simulink model "fft_biplex_real_4x_dsp48_opt_test"  (Simulink 7.4)
settings: Solver=VariableStepDiscrete  StartTime=0.0  StopTime=128  RelTol=1e-3
libraries: xbsIndex_r4 x620, casper_library_misc x24, casper_library_delays x6, casper_library_ffts_twiddle x1, simulink x1
(part 1 of 7)
settings Model: Creator=User  LastModifiedBy=wjm
settings OptimizationCC: InitFltsAndDblsToZero=on
settings DebuggingCC: SaveWithDisabledLinksMsg=none  SaveWithParameterizedLinksMsg=none

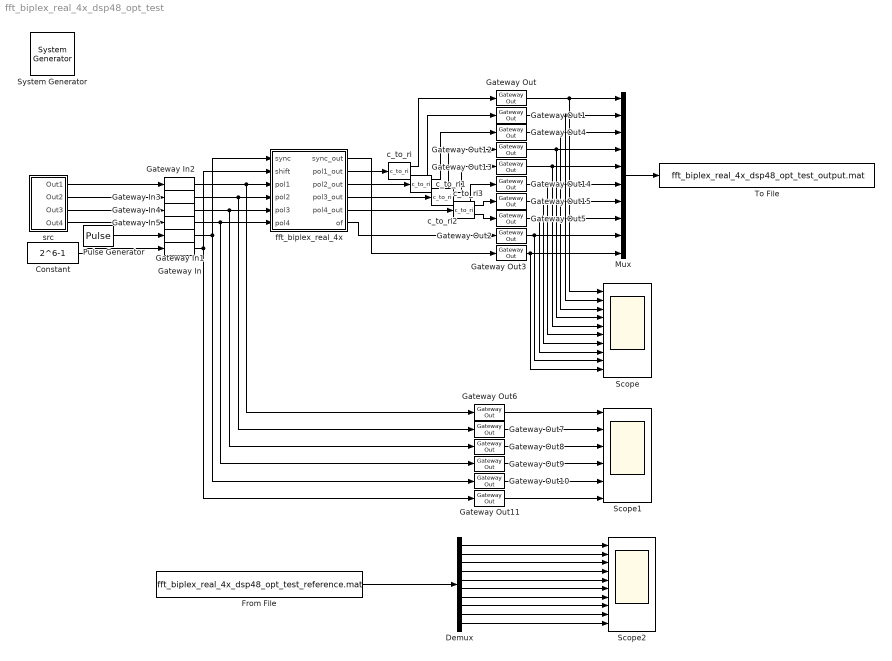
== system fft_biplex_real_4x_dsp48_opt_test ==
  " System Generator" : xbsIndex_r4/ System Generator  Tag=genX  SystemSampleTime=-1  xilinxfamily=virtex5  part=xc5vsx95t  speed=-1  package=ff1136  synthesis_tool=XST  clock_wrapper=Clock Enables  directory=./netlist  testbench=off  simulink_period=1  sysclk_period=100  dcm_input_clock_period=100  incr_netlist=off  trim_vbits=Everywhere in SubSystem  dbl_ovrd=According to Block Masks  core_generation=According to Block Masks  run_coregen=off  deprecated_control=off  eval_field=0  block_type=sysgen
      settings: block_version=10.1.1
  Constant : Constant  Value=2^6-1  OutDataType=sfix(16)  OutScaling=2^0
  Demux : Demux  Outputs=10
  From File : FromFile  FileName=fft_biplex_real_4x_dsp48_opt_test_reference.mat  SampleTime=1
  Gateway In : xbsIndex_r4/Gateway In  arith_type=Unsigned  n_bits=6  bin_pt=0  quantization=Truncate  overflow=Wrap  period=1  dbl_ovrd=off  timing_constraint=None  locs_specified=off  LOCs={}  hdl_port=on  block_type=gatewayin
      settings: infoedit="Gateway in block.  Converts inputs of type Simulink integer, double and fixed point to  Xilinx fixed point type.<P><P>Hardware notes:  In hardware these blocks become top level input ports."  block_version=10.1.1
  Gateway In1 : xbsIndex_r4/Gateway In  arith_type=Boolean  n_bits=16  bin_pt=14  quantization="Round  (unbiased: +/- Inf)"  overflow=Saturate  period=1  dbl_ovrd=off  timing_constraint=None  locs_specified=off  LOCs={}  hdl_port=on  block_type=gatewayin
      settings: infoedit="Gateway in block.  Converts inputs of type Simulink integer, double and fixed point to  Xilinx fixed point type.<P><P>Hardware notes:  In hardware these blocks become top level input ports."  block_version=10.1.1
  Gateway In{2..5} (4 alike) : xbsIndex_r4/Gateway In  arith_type="Signed  (2's comp)"  n_bits=8  bin_pt=7  quantization=Truncate  overflow=Wrap  period=1  dbl_ovrd=off  timing_constraint=None  locs_specified=off  LOCs={}  hdl_port=on  block_type=gatewayin
      settings: infoedit="Gateway in block.  Converts inputs of type Simulink integer, double and fixed point to  Xilinx fixed point type.<P><P>Hardware notes:  In hardware these blocks become top level input ports."  block_version=10.1.1
  Gateway Out{,1..15} (16 alike) : xbsIndex_r4/Gateway Out  hdl_port=on  timing_constraint=None  locs_specified=off  LOCs={}  block_type=gatewayout
      settings: infoedit="Gateway out block.  Converts Xilinx fixed point inputs into ouputs of type Simulink integer, double, or fixed point.<P><P>Hardware notes:  In hardware these blocks become top level output ports or are discarded, depending on how they are configured."  block_version=10.1.1
  Mux : Mux  Inputs=10
  Pulse Generator : DiscretePulseGenerator  Amplitude=1  Period=2^5  PulseWidth=1  PhaseDelay=13  SampleTime=1
  Scope : Scope  NumInputPorts=10
      settings: TimeRange=256  YMin=-5~-5~-5~-5~-1~-5~-5~-5~-5~-5  YMax=5~5~5~5~2~5~5~5~5~5
  Scope1 : Scope  NumInputPorts=6
      settings: YMin=-5~-5~-5~-5~-5~-5  YMax=5~5~5~5~5~5
  Scope2 : Scope  NumInputPorts=10
      settings: TimeRange=256  YMin=-5~-5~-5~-5~-1~-5~-5~-5~-5~-5  YMax=5~5~5~5~2~5~5~5~5~5  SaveName=ScopeData2
  To File : ToFile  Filename=fft_biplex_real_4x_dsp48_opt_test_output.mat  MatrixName=output
  c_to_ri{,1..3} (4 alike) : casper_library_misc/c_to_ri  SystemSampleTime=-1  n_bits=8  bin_pt=7
      settings: AttributesFormatString=8_7 r/i
  fft_biplex_real_4x : Subsystem  AncestorBlock=casper_library_ffts/fft_biplex_real_4x  mask(fft_biplex_real_4x){FFTSize=3, input_bit_width=8, coeff_bit_width=8, add_latency=2, mult_latency=3, bram_latency=1, conv_latency=1, quantization=Truncate, overflow=Wrap, arch=Virtex5, opt_target=logic, coeffs_bit_limit=8, delays_bit_limit=8, specify_mult=on, mult_spec=[0                                      1                                      2], hardcode_shifts=off, shift_schedule=getfield( getfield( get_param( gcb,'UserData' ), 'parameters'),'shift_schedule'), dsp48_adders=on}
      mask prompts: FFTSize "Size of FFT: (2^? pts)"; input_bit_width "Input/Output Bit Width"; coeff_bit_width "Coefficient Bit Width"; add_latency "Add Latency"; mult_latency "Mult Latency"; bram_latency "BRAM Latency"; conv_latency "Convert latency"; quantization "Quantization Behavior"; overflow "Overflow Behavior"; arch "Architecture"; opt_target "Use less"; coeffs_bit_limit "Number bits above which to store stage's coefficients in BRAM (2^? bits)"; delays_bit_limit "Number bits above which to implement stage's delays in BRAM (2^? bits)"; specify_mult "Specify multiplier use (behavioral HDL if not specified)"; mult_spec "Multiplier specification (0=core, 1=embedded, 2=behavioural) (left=1st stage)"; hardcode_shifts "Hardcode shift schedule"; shift_schedule "Shift schedule"; dsp48_adders "DSP48 adders in butterfly"
      mask help: A real-sampled biplex FFT, with output demuxed by 4.
      mask init:
      | fft_biplex_real_4x_init(gcb, ...
      |     'FFTSize', FFTSize, ...
      |     'input_bit_width', input_bit_width, ...
      |     'coeff_bit_width', coeff_bit_width, ...
      |     'add_latency', add_latency, ...
      |     'mult_latency', mult_latency, ...
      |     'bram_latency', bram_latency, ...
      |     'conv_latency', conv_latency, ...
      |     'quantization', quantization, ...
      |     'overflow', overflow, ...
      |     'arch', arch, ...
      |     'opt_target', opt_target, ...
      |     'coeffs_bit_limit', coeffs_bit_limit, ...
      |     'delays_bit_limit', delays_bit_limit, ...    
      |     'specify_mult', specify_mult, ...
      |     'mult_spec', mult_spec, ...
      |     'hardcode_shifts', hardcode_shifts, ...
      |     'shift_schedule', shift_schedule, ...
      |     'dsp48_adders', dsp48_adders);
      settings: AttributesFormatString=|
      | Virtex5
      | 3 stages
      | [8,8]
      | Truncate
      | Wrap
      mask Help: eval('xlWeb(''http://casper.berkeley.edu/wiki/Fft_biplex_real_4x'')')
      mask StyleString: edit,edit,edit,edit,edit,edit,edit,popup(Truncate|Round  (unbiased: +/- Inf)|Round  (unbiased: Even Values)),popup(Wrap|Saturate|Error),popup(Virtex2Pro|Virtex5),popup(logic|multipliers),edit,edit,checkbox,edit,checkbox,edit,checkbox
      mask CallbackString:
      | |||||||||fft_callback_arch(gcb);||||specify_mult = get_param(gcb, 'specify_mult');
      | set_param_state(gcb, 'mult_spec', specify_mult);||hardcode_shifts = get_param(gcb, 'hardcode_shifts');
      | set_param_state(gcb, 'shift_schedule', hardcode_shifts);||fft_callback_dsp48_adders(gcb);
      mask TabNameString: Basic,Basic,Basic,Latency,Latency,Latency,Latency,Implementation,Implementation,Implementation,Implementation,Implementation,Implementation,Implementation,Implementation,Implementation,Implementation,Implementation
  src : Subsystem
  wires:
  Gateway In/1 -> Gateway Out11/1, fft_biplex_real_4x/2(shift)
  Pulse Generator/1 -> Gateway In1/1
  Gateway In1/1 -> Gateway Out10/1, fft_biplex_real_4x/1(sync)
  src/1(Out1) -> Gateway In2/1
  src/2(Out2) -> Gateway In3/1
  src/3(Out3) -> Gateway In4/1
  src/4(Out4) -> Gateway In5/1
  Gateway In2/1 -> Gateway Out6/1, fft_biplex_real_4x/3(pol1)
  Gateway In3/1 -> Gateway Out7/1, fft_biplex_real_4x/4(pol2)
  Gateway In4/1 -> Gateway Out8/1, fft_biplex_real_4x/5(pol3)
  Gateway In5/1 -> Gateway Out9/1, fft_biplex_real_4x/6(pol4)
  Gateway Out6/1 -> Scope1/1
  Gateway Out7/1 -> Scope1/2
  Gateway Out8/1 -> Scope1/3
  Gateway Out9/1 -> Scope1/4
  Gateway Out10/1 -> Scope1/5
  Gateway Out11/1 -> Scope1/6
  Constant/1 -> Gateway In/1
  Mux/1 -> To File/1
  c_to_ri/1 -> Gateway Out/1
  c_to_ri/2 -> Gateway Out1/1
  c_to_ri1/1 -> Gateway Out4/1
  c_to_ri1/2 -> Gateway Out12/1
  c_to_ri2/1 -> Gateway Out13/1
  c_to_ri2/2 -> Gateway Out14/1
  c_to_ri3/1 -> Gateway Out15/1
  c_to_ri3/2 -> Gateway Out5/1
  Gateway Out/1 -> Scope/1, Mux/1
  Gateway Out1/1 -> Scope/2, Mux/2
  Gateway Out4/1 -> Scope/3, Mux/3
  Gateway Out12/1 -> Scope/4, Mux/4
  Gateway Out13/1 -> Scope/5, Mux/5
  Gateway Out14/1 -> Scope/6, Mux/6
  Gateway Out15/1 -> Scope/7, Mux/7
  Gateway Out5/1 -> Scope/8, Mux/8
  Gateway Out2/1 -> Scope/9, Mux/9
  Gateway Out3/1 -> Scope/10, Mux/10
  Demux/1 -> Scope2/1
  Demux/2 -> Scope2/2
  Demux/3 -> Scope2/3
  Demux/4 -> Scope2/4
  Demux/5 -> Scope2/5
  Demux/6 -> Scope2/6
  Demux/7 -> Scope2/7
  Demux/8 -> Scope2/8
  Demux/9 -> Scope2/9
  Demux/10 -> Scope2/10
  From File/1 -> Demux/1
  fft_biplex_real_4x/2(pol1_out) -> c_to_ri/1
  fft_biplex_real_4x/3(pol2_out) -> c_to_ri1/1
  fft_biplex_real_4x/4(pol3_out) -> c_to_ri2/1
  fft_biplex_real_4x/5(pol4_out) -> c_to_ri3/1
  fft_biplex_real_4x/6(of) -> Gateway Out2/1
  fft_biplex_real_4x/1(sync_out) -> Gateway Out3/1

== system fft_biplex_real_4x_dsp48_opt_test/fft_biplex_real_4x ==
  sync : Inport  OutDataType=sfix(16)  OutScaling=2^0
  shift : Inport  Port=2  OutDataType=sfix(16)  OutScaling=2^0
  pol1 : Inport  Port=3  OutDataType=sfix(16)  OutScaling=2^0
  pol2 : Inport  Port=4  OutDataType=sfix(16)  OutScaling=2^0
  pol3 : Inport  Port=5  OutDataType=sfix(16)  OutScaling=2^0
  pol4 : Inport  Port=6  OutDataType=sfix(16)  OutScaling=2^0
  bi_real_unscr_4x : Subsystem  AncestorBlock=casper_library_ffts_internal/bi_real_unscr_4x  mask(bi_real_unscr_4x){FFTSize=3, n_bits=8, add_latency=2, conv_latency=1, bram_latency=1, bram_map=off, bram_delays=off, dsp48_adders=on}
      mask prompts: FFTSize "Size of FFT (2^?):"; n_bits "Sample Bit Width"; add_latency "Add Latency"; conv_latency "Convert Latency"; bram_latency "BRAM Latency"; bram_map "Use BlockRAM for Map"; bram_delays "Use BlockRAM for Delays"; dsp48_adders "Use DSP48s for adders"
      mask help: FFT internal block.
      mask init:
      | bi_real_unscr_4x_init(gcb, ...
      |     'FFTSize', FFTSize, ...
      |     'n_bits', n_bits, ...
      |     'add_latency', add_latency, ...
      |     'conv_latency', conv_latency, ...
      |     'bram_latency', bram_latency, ...
      |     'bram_map', bram_map, ...
      |     'bram_delays', bram_delays, ...
      |     'dsp48_adders', dsp48_adders);
      mask TabNameString: Basic,Basic,Latency,Latency,Latency,Implementation,Implementation,Implementation
  biplex_core : Subsystem  AncestorBlock=casper_library_ffts/biplex_core  mask(biplex_core){FFTSize=3, input_bit_width=8, coeff_bit_width=8, add_latency=2, mult_latency=3, bram_latency=1, conv_latency=1, quantization=Truncate, overflow=Wrap, arch=Virtex5, opt_target=logic, coeffs_bit_limit=8, delays_bit_limit=8, specify_mult=on, mult_spec=[0                                      1                                      2], hardcode_shifts=off, shift_schedule=getfield( getfield( get_param( gcb,'UserData' ), 'parameters'),'shift_schedule'), dsp48_adders=on}
      mask prompts: FFTSize "Size of FFT: (2^? pts)"; input_bit_width "Input/Output Bit Width"; coeff_bit_width "Coefficient Bit Width"; add_latency "Add Latency"; mult_latency "Mult Latency"; bram_latency "BRAM Latency"; conv_latency "Convert latency"; quantization "Quantization Behavior"; overflow "Overflow Behavior"; arch "Architecture"; opt_target "Use less"; coeffs_bit_limit "Number bits above which to store stage's coefficients in BRAM (2^? bits)"; delays_bit_limit "Number bits above which to implent stage's delays in BRAM (2^? bits)"; specify_mult "Specify multiplier use (behavioural HDL if not specified)"; mult_spec "Multiplier specification (0=core, 1=embedded, 2=behavioural) (left=1st stage)"; hardcode_shifts "Hardcode shift schedule"; shift_schedule "Shift schedule"; dsp48_adders "Use DSP48s for adders"
      mask help: FFT internal block.
      mask init:
      | biplex_core_init(gcb,...
      |     'FFTSize', FFTSize,...
      |     'input_bit_width', input_bit_width,...
      |     'coeff_bit_width', coeff_bit_width,...
      |     'add_latency', add_latency,...
      |     'mult_latency', mult_latency,...
      |     'bram_latency', bram_latency,...
      |     'conv_latency', conv_latency, ...
      |     'quantization', quantization,...
      |     'overflow', overflow,...
      |     'arch', arch, ...
      |     'opt_target', opt_target, ...
      |     'coeffs_bit_limit', coeffs_bit_limit, ...
      |     'delays_bit_limit', delays_bit_limit, ...
      |     'specify_mult', specify_mult, ...
      |     'mult_spec', mult_spec, ...
      |     'hardcode_shifts', hardcode_shifts, ...
      |     'shift_schedule', shift_schedule, ...
      |     'dsp48_adders', dsp48_adders );
      settings: AttributesFormatString=|
      | 3 stages
      | reduce logic
      | Virtex5
      mask StyleString: edit,edit,edit,edit,edit,edit,edit,popup(Truncate|Round  (unbiased: +/- Inf)|Round  (unbiased: Even Values)),popup(Wrap|Saturate|Error),popup(Virtex2Pro|Virtex5),popup(logic|multipliers),edit,edit,checkbox,edit,checkbox,edit,checkbox
      mask CallbackString:
      | |||||||||fft_callback_arch(gcb);||||specify_mult = get_param(gcb, 'specify_mult');
      | set_param_state(gcb, 'mult_spec', specify_mult);||hardcode_shifts = get_param(gcb, 'hardcode_shifts');
      | set_param_state(gcb, 'shift_schedule', hardcode_shifts);||fft_callback_dsp48_adders(gcb);
      mask TabNameString: Basic,Basic,Basic,Latency,Latency,Latency,Latency,Implementation,Implementation,Implementation,Implementation,Implementation,Implementation,Implementation,Implementation,Implementation,Implementation,Implementation
  ri_to_c0 : Subsystem  AncestorBlock=casper_library_misc/ri_to_c
      mask Type: ri_to_c
      mask Description:
      | Concatenates real and imaginary inputs into a complex output.
      | Useful for simplifying interconnects.
      | See also: Complex to Real-Imag (c_to_ri)
      mask Help: eval('xlWeb(''http://casper.berkeley.edu/wiki/Ri_to_c'')')
  ri_to_c1 : Subsystem  AncestorBlock=casper_library_misc/ri_to_c
      mask Type: ri_to_c
      mask Description:
      | Concatenates real and imaginary inputs into a complex output.
      | Useful for simplifying interconnects.
      | See also: Complex to Real-Imag (c_to_ri)
      mask Help: eval('xlWeb(''http://casper.berkeley.edu/wiki/Ri_to_c'')')
  sync_out : Outport  OutDataType=sfix(16)  OutScaling=2^0
  pol1_out : Outport  Port=2  OutDataType=sfix(16)  OutScaling=2^0
  pol2_out : Outport  Port=3  OutDataType=sfix(16)  OutScaling=2^0
  pol3_out : Outport  Port=4  OutDataType=sfix(16)  OutScaling=2^0
  pol4_out : Outport  Port=5  OutDataType=sfix(16)  OutScaling=2^0
  of : Outport  Port=6  OutDataType=sfix(16)  OutScaling=2^0
  wires:
  pol1/1 -> ri_to_c0/1(re)
  pol2/1 -> ri_to_c0/2(im)
  pol3/1 -> ri_to_c1/1(re)
  pol4/1 -> ri_to_c1/2(im)
  sync/1 -> biplex_core/1(sync)
  shift/1 -> biplex_core/2(shift)
  ri_to_c0/1(c) -> biplex_core/3(pol1)
  ri_to_c1/1(c) -> biplex_core/4(pol2)
  biplex_core/1(sync_out) -> bi_real_unscr_4x/1(sync)
  biplex_core/2(out1) -> bi_real_unscr_4x/2(even)
  biplex_core/3(out2) -> bi_real_unscr_4x/3(odd)
  biplex_core/4(of) -> of/1
  bi_real_unscr_4x/1(sync_out) -> sync_out/1
  bi_real_unscr_4x/2(pol1_out) -> pol1_out/1
  bi_real_unscr_4x/3(pol2_out) -> pol2_out/1
  bi_real_unscr_4x/4(pol3_out) -> pol3_out/1
  bi_real_unscr_4x/5(pol4_out) -> pol4_out/1

== system fft_biplex_real_4x_dsp48_opt_test/src ==
  Band-Limited White Noise : simulink/Sources/Band-Limited White Noise  SystemSampleTime=-1  Cov=[0.001]  Ts=1  seed=[23341]
  Constant : Constant  Value=0  OutDataType=sfix(16)  OutScaling=2^0
  Pulse Generator1 : DiscretePulseGenerator  Amplitude=0.75  Period=2^4  PulseWidth=1  PhaseDelay=15  SampleTime=1
  Pulse Generator2 : DiscretePulseGenerator  Amplitude=0.75  Period=2^3  PulseWidth=1  PhaseDelay=16  SampleTime=1
  Sine Wave : Sin  SineType=Sample based  Amplitude=0.1  Bias=0  Frequency=1  Phase=0  Samples=8  SampleTime=1  Offset=0
  Out1 : Outport
  Out2 : Outport  Port=2
  Out3 : Outport  Port=3
  Out4 : Outport  Port=4
  wires:
  Pulse Generator1/1 -> Out1/1
  Constant/1 -> Out3/1
  Sine Wave/1 -> Out2/1
  Band-Limited White Noise/1 -> Out4/1

== system fft_biplex_real_4x_dsp48_opt_test/fft_biplex_real_4x/bi_real_unscr_4x ==
  sync : Inport
  even : Inport  Port=2
  odd : Inport  Port=3
  Constant0 : xbsIndex_r4/Constant  arith_type=Unsigned  const=2^(FFTSize-1)  n_bits=FFTSize  bin_pt=0  explicit_period=on  period=1  equ=P=C  opselect=C  inp2=PCIN>>17  opr=+  inp1=P  carry=CIN  dbl_ovrd=off  block_type=constant
      settings: block_version=11.4
  Constant1 : xbsIndex_r4/Constant  arith_type=Unsigned  const=0  n_bits=FFTSize  bin_pt=0  explicit_period=on  period=1  equ=P=C  opselect=C  inp2=PCIN>>17  opr=+  inp1=P  carry=CIN  dbl_ovrd=off  block_type=constant
      settings: block_version=11.4
  Counter0 : xbsIndex_r4/Counter  cnt_type=Free Running  cnt_to=Inf  operation=Up  start_count=0  cnt_by_val=1  arith_type=Unsigned  n_bits=FFTSize  bin_pt=0  load_pin=off  rst=on  en=off  explicit_period=on  period=1  dbl_ovrd=off  use_behavioral_HDL=off  implementation=Fabric  block_type=counter
      settings: block_version=11.4
  Delay : xbsIndex_r4/Delay  en=off  latency=1  dbl_ovrd=off  reg_retiming=off  block_type=delay
      settings: block_version=11.4
  Mux{0..3} (4 alike) : xbsIndex_r4/Mux  inputs=2  en=off  latency=1  precision=Full  arith_type=Unsigned  n_bits=16  bin_pt=14  quantization=Truncate  overflow=Wrap  dbl_ovrd=off  block_type=mux
      settings: block_version=11.4
  Relational0 : xbsIndex_r4/Relational  mode=a=b  en=off  latency=0  dbl_ovrd=off  block_type=relational
  Relational1 : xbsIndex_r4/Relational  mode=a=b  en=off  latency=0  dbl_ovrd=off  block_type=relational
  delay_srl0 : Subsystem  AncestorBlock=casper_library_delays/delay_srl  mask(delay_srl){DelayLen=2^(FFTSize-1)}
      mask prompts: DelayLen "Delay by:"
      mask help:
      | A delay block that uses slices (SRL16s) for its storage.
      |
      | It explicitly converts the first delay into a flip flop,
      | and lets XSG break up the remaining delays into a series
      | of SRL16+FF instances.
      |
      | This is advantageous because the setup time of an SRL is
      | longer than that of a flip flop.
      mask init:
      | if (DelayLen > 0),
      |     ff_delay = 1;
      |     srl_delay = DelayLen - 1;
      | else
      |     ff_delay = 0;
      |     srl_delay = 0;
      | end
      mask Help: eval('xlWeb(''http://casper.berkeley.edu/wiki/Delay_srl'')')
  delay_srl1 : Subsystem  AncestorBlock=casper_library_delays/delay_srl  mask(delay_srl){DelayLen=2^(FFTSize-1)}
      mask prompts: DelayLen "Delay by:"
      mask help:
      | A delay block that uses slices (SRL16s) for its storage.
      |
      | It explicitly converts the first delay into a flip flop,
      | and lets XSG break up the remaining delays into a series
      | of SRL16+FF instances.
      |
      | This is advantageous because the setup time of an SRL is
      | longer than that of a flip flop.
      mask init:
      | if (DelayLen > 0),
      |     ff_delay = 1;
      |     srl_delay = DelayLen - 1;
      | else
      |     ff_delay = 0;
      |     srl_delay = 0;
      | end
      mask Help: eval('xlWeb(''http://casper.berkeley.edu/wiki/Delay_srl'')')
  en_even : xbsIndex_r4/Constant  arith_type=Boolean  const=1  n_bits=1  bin_pt=0  explicit_period=on  period=1  equ=P=C  opselect=C  inp2=PCIN>>17  opr=+  inp1=P  carry=CIN  dbl_ovrd=off  block_type=constant
      settings: block_version=11.4
  en_odd : xbsIndex_r4/Constant  arith_type=Boolean  const=1  n_bits=1  bin_pt=0  explicit_period=on  period=1  equ=P=C  opselect=C  inp2=PCIN>>17  opr=+  inp1=P  carry=CIN  dbl_ovrd=off  block_type=constant
      settings: block_version=11.4
  en_out : xbsIndex_r4/Constant  arith_type=Boolean  const=1  n_bits=1  bin_pt=0  explicit_period=on  period=1  equ=P=C  opselect=C  inp2=PCIN>>17  opr=+  inp1=P  carry=CIN  dbl_ovrd=off  block_type=constant
      settings: block_version=11.4
  hilbert_dsp48e0 : Subsystem  AncestorBlock=casper_library_ffts_internal/hilbert_dsp48e  mask(sincos_dsp48e){BitWidth=n_bits, conv_latency=conv_latency}
      mask prompts: BitWidth "Bit Wdith"; conv_latency "Convert Latency"
      mask help:
      | FFT internal block.
      |
      | Computes (a+b*)/2 and (a-b*)/2i.
  hilbert_dsp48e1 : Subsystem  AncestorBlock=casper_library_ffts_internal/hilbert_dsp48e  mask(sincos_dsp48e){BitWidth=n_bits, conv_latency=conv_latency}
      mask prompts: BitWidth "Bit Wdith"; conv_latency "Convert Latency"
      mask help:
      | FFT internal block.
      |
      | Computes (a+b*)/2 and (a-b*)/2i.
  mirror_spectrum : Subsystem  AncestorBlock=casper_library_ffts_internal/mirror_spectrum  mask(mirror_spectrum){FFTSize=3, input_bitwidth=8, bram_latency=1, negate_latency=1}
      mask prompts: FFTSize "Size of FFT (2^?)"; input_bitwidth "Input Bit Width"; bram_latency "BRAM Latency"; negate_latency "Negate Latency"
      mask help: FFT internal block.
      mask TabNameString: Basic,Basic,Latency,Latency
  reorder_even : Subsystem  AncestorBlock=casper_library_reorder/reorder  mask(reorder){map=[0 2 1 3], n_inputs=1, bram_latency=bram_latency, map_latency=0, double_buffer=0, bram_map=off}
      mask prompts: map "Output Order:"; n_inputs "Number of inputs"; bram_latency "BRAM Latency"; map_latency "Map Latency"; double_buffer "Double Buffer"; bram_map "Use BlockRAM for Map"
      mask init:
      | reorder_init(gcb, ...
      |     'map', map, ...
      |     'n_inputs', n_inputs, ...
      |     'bram_latency', bram_latency, ...
      |     'map_latency', map_latency, ...
      |     'double_buffer', double_buffer, ...
      |     'bram_map', bram_map);
      settings: AttributesFormatString=order=2
      mask Help: eval('xlWeb(''http://casper.berkeley.edu/wiki/Reorder'')')
  reorder_odd : Subsystem  AncestorBlock=casper_library_reorder/reorder  mask(reorder){map=[3 1 2 0], n_inputs=1, bram_latency=bram_latency, map_latency=0, double_buffer=0, bram_map=off}
      mask prompts: map "Output Order:"; n_inputs "Number of inputs"; bram_latency "BRAM Latency"; map_latency "Map Latency"; double_buffer "Double Buffer"; bram_map "Use BlockRAM for Map"
      mask init: same as fft_biplex_real_4x_dsp48_opt_test/fft_biplex_real_4x/bi_real_unscr_4x/reorder_even
      settings: AttributesFormatString=order=2
      mask Help: eval('xlWeb(''http://casper.berkeley.edu/wiki/Reorder'')')
  reorder_out : Subsystem  AncestorBlock=casper_library_reorder/reorder  mask(reorder){map=[3 2 1 0], n_inputs=4, bram_latency=bram_latency, map_latency=0, double_buffer=0, bram_map=off}
      mask prompts: map "Output Order:"; n_inputs "Number of inputs"; bram_latency "BRAM Latency"; map_latency "Map Latency"; double_buffer "Double Buffer"; bram_map "Use BlockRAM for Map"
      mask init: same as fft_biplex_real_4x_dsp48_opt_test/fft_biplex_real_4x/bi_real_unscr_4x/reorder_even
      settings: AttributesFormatString=order=2
      mask Help: eval('xlWeb(''http://casper.berkeley.edu/wiki/Reorder'')')
  sync_delay_srl : Subsystem  AncestorBlock=casper_library_delays/delay_srl  mask(delay_srl){DelayLen=2^(FFTSize-1) + add_latency + conv_latency + 1}
      mask prompts: DelayLen "Delay by:"
      mask help:
      | A delay block that uses slices (SRL16s) for its storage.
      |
      | It explicitly converts the first delay into a flip flop,
      | and lets XSG break up the remaining delays into a series
      | of SRL16+FF instances.
      |
      | This is advantageous because the setup time of an SRL is
      | longer than that of a flip flop.
      mask init:
      | if (DelayLen > 0),
      |     ff_delay = 1;
      |     srl_delay = DelayLen - 1;
      | else
      |     ff_delay = 0;
      |     srl_delay = 0;
      | end
      mask Help: eval('xlWeb(''http://casper.berkeley.edu/wiki/Delay_srl'')')
  sync_out : Outport
  pol1_out : Outport  Port=2
  pol2_out : Outport  Port=3
  pol3_out : Outport  Port=4
  pol4_out : Outport  Port=5
  wires:
  sync/1 -> reorder_even/1(sync), reorder_odd/1(sync)
  en_even/1 -> reorder_even/2(en)
  even/1 -> reorder_even/3(din0)
  en_odd/1 -> reorder_odd/2(en)
  odd/1 -> reorder_odd/3(din0)
  reorder_odd/3(dout0) -> Delay/1
  reorder_even/1(sync_out) -> Counter0/1, sync_delay_srl/1(in)
  Constant0/1 -> Relational0/1
  Counter0/1 -> Relational0/2, Relational1/1
  Constant1/1 -> Relational1/2
  Relational0/1 -> Mux0/1, Mux3/1
  Relational1/1 -> Mux1/1, Mux2/1
  reorder_even/3(dout0) -> Mux0/2, Mux1/3, Mux2/2, Mux3/3
  Delay/1 -> Mux0/3, Mux1/2, Mux2/3, Mux3/2
  Mux0/1 -> hilbert_dsp48e0/1(a)
  Mux1/1 -> hilbert_dsp48e0/2(b)
  Mux2/1 -> hilbert_dsp48e1/1(a)
  Mux3/1 -> hilbert_dsp48e1/2(b)
  hilbert_dsp48e0/1(even) -> delay_srl0/1(in)
  hilbert_dsp48e0/2(odd) -> delay_srl1/1(in)
  sync_delay_srl/1(out) -> reorder_out/1(sync), mirror_spectrum/1(sync)
  en_out/1 -> reorder_out/2(en)
  delay_srl0/1(out) -> reorder_out/3(din0), mirror_spectrum/2(din0)
  delay_srl1/1(out) -> reorder_out/4(din1), mirror_spectrum/4(din1)
  hilbert_dsp48e1/1(even) -> reorder_out/5(din2), mirror_spectrum/6(din2)
  hilbert_dsp48e1/2(odd) -> reorder_out/6(din3), mirror_spectrum/8(din3)
  reorder_out/3(dout0) -> mirror_spectrum/3(reo_in0)
  reorder_out/4(dout1) -> mirror_spectrum/5(reo_in1)
  reorder_out/5(dout2) -> mirror_spectrum/7(reo_in2)
  reorder_out/6(dout3) -> mirror_spectrum/9(reo_in3)
  mirror_spectrum/1(sync_out) -> sync_out/1
  mirror_spectrum/2(dout0) -> pol1_out/1
  mirror_spectrum/3(dout1) -> pol2_out/1
  mirror_spectrum/4(dout2) -> pol3_out/1
  mirror_spectrum/5(dout3) -> pol4_out/1

== system fft_biplex_real_4x_dsp48_opt_test/fft_biplex_real_4x/biplex_core ==
  sync : Inport
  shift : Inport  Port=2
  pol1 : Inport  Port=3
  pol2 : Inport  Port=4
  Constant : xbsIndex_r4/Constant  arith_type=Boolean  const=0  n_bits=16  bin_pt=14  explicit_period=off  period=1  equ=P=C  opselect=C  inp2=PCIN>>17  opr=+  inp1=P  carry=CIN  dbl_ovrd=off  block_type=constant
      settings: block_version=11.4
  fft_stage_1 : Subsystem  AncestorBlock=casper_library_ffts/fft_stage_n  mask(fft_stage_n){FFTSize=3, FFTStage=1, input_bit_width=8, coeff_bit_width=8, downshift=off, add_latency=2, mult_latency=3, bram_latency=1, conv_latency=1, quantization=Truncate, overflow=Wrap, arch=Virtex5, opt_target=logic, delays_bram=off, coeffs_bram=off, use_hdl=on, use_embedded=off, hardcode_shifts=off, dsp48_adders=on}
      mask prompts: FFTSize "Size of FFT: (2^? pts)"; FFTStage "Stage of FFT:"; input_bit_width "Input/Output Bit Width:"; coeff_bit_width "Coefficient Bit Width"; add_latency "Add Latency"; mult_latency "Mult Latency"; bram_latency "BRAM Latency"; conv_latency "Convert latency"; quantization "Quantization Behavior"; overflow "Overflow Behavior"; arch "Architecture"; opt_target "Use less"; delays_bram "Implement Delays in BRAM"; coeffs_bram "Store Coefficients in BRAM"; use_hdl "Use behavioural HDL for mutlipliers"; use_embedded "Use embedded multipliers"; hardcode_shifts "Hardcode shift schedule"; dsp48_adders "Use DSP48s for adders"
      mask help: FFT internal block.
      mask init:
      | fft_stage_n_init(gcb, ...
      |     'FFTSize', FFTSize, ...
      |     'FFTStage', FFTStage, ...
      |     'input_bit_width', input_bit_width, ...
      |     'coeff_bit_width', coeff_bit_width, ...
      |     'delays_bram', delays_bram, ...
      |     'coeffs_bram', coeffs_bram, ...
      |     'quantization', quantization, ...
      |     'overflow', overflow, ...
      |     'add_latency', add_latency, ...
      |     'mult_latency', mult_latency, ...
      |     'bram_latency', bram_latency, ...
      |     'conv_latency', conv_latency, ...
      |     'arch', arch, ...
      |     'opt_target', opt_target, ...
      |     'use_hdl', use_hdl, ...
      |     'use_embedded', use_embedded, ...
      |     'hardcode_shifts', hardcode_shifts, ...
      |     'downshift', downshift, ...
      |     'dsp48_adders', dsp48_adders);
      settings: AttributesFormatString=|
      | [1/3]
      | delays in slices
      | coeffs in slices
      mask StyleString: edit,edit,edit,edit,checkbox,edit,edit,edit,edit,popup(Truncate|Round  (unbiased: +/- Inf)|Round  (unbiased: Even Values)),popup(Wrap|Saturate|Error),popup(Virtex2Pro|Virtex5),popup(logic|multipliers),checkbox,checkbox,checkbox,checkbox,checkbox,checkbox
      mask CallbackString:
      | |||||||||||fft_callback_arch(gcb);||||% make mutually exclusive with use_embedded.
      | 
      | use_hdl = get_param(gcb, 'use_hdl');
      | if strcmp(use_hdl, 'on'),
      |     set_param_state(gcb, 'use_embedded', 'off');
      | else
      |     set_param_state(gcb, 'use_embedded', 'on');
      | end|% make mutually exclusive with use_hdl.
      | 
      | use_hdl = get_param(gcb, 'use_embedded');
      | if strcmp(use_hdl, 'on'),
      |     set_param_state(gcb, 'use_hdl', 'off');
      | else
      |     set_param_state(gcb, 'use_hdl', 'on');
      | end|hardcode_shifts = get_param(gcb, 'hardcode_shifts');
      | set_param_state(gcb, 'downshift', hardcode_shifts);|fft_callback_dsp48_adders(gcb);
      mask TabNameString: Basic,Basic,Basic,Basic,Basic,Latency,Latency,Latency,Latency,Implementation,Implementation,Implementation,Implementation,Implementation,Implementation,Implementation,Implementation,Implementation,Implementation
  fft_stage_2 : Subsystem  AncestorBlock=casper_library_ffts/fft_stage_n  mask(fft_stage_n){FFTSize=3, FFTStage=2, input_bit_width=8, coeff_bit_width=8, downshift=off, add_latency=2, mult_latency=3, bram_latency=1, conv_latency=1, quantization=Truncate, overflow=Wrap, arch=Virtex5, opt_target=logic, delays_bram=off, coeffs_bram=off, use_hdl=off, use_embedded=on, hardcode_shifts=off, dsp48_adders=on}
      mask prompts: FFTSize "Size of FFT: (2^? pts)"; FFTStage "Stage of FFT:"; input_bit_width "Input/Output Bit Width:"; coeff_bit_width "Coefficient Bit Width"; add_latency "Add Latency"; mult_latency "Mult Latency"; bram_latency "BRAM Latency"; conv_latency "Convert latency"; quantization "Quantization Behavior"; overflow "Overflow Behavior"; arch "Architecture"; opt_target "Use less"; delays_bram "Implement Delays in BRAM"; coeffs_bram "Store Coefficients in BRAM"; use_hdl "Use behavioural HDL for mutlipliers"; use_embedded "Use embedded multipliers"; hardcode_shifts "Hardcode shift schedule"; dsp48_adders "Use DSP48s for adders"
      mask help: FFT internal block.
      mask init: same as fft_biplex_real_4x_dsp48_opt_test/fft_biplex_real_4x/biplex_core/fft_stage_1
      settings: AttributesFormatString=|
      | [2/3]
      | delays in slices
      | coeffs in slices
      mask StyleString: edit,edit,edit,edit,checkbox,edit,edit,edit,edit,popup(Truncate|Round  (unbiased: +/- Inf)|Round  (unbiased: Even Values)),popup(Wrap|Saturate|Error),popup(Virtex2Pro|Virtex5),popup(logic|multipliers),checkbox,checkbox,checkbox,checkbox,checkbox,checkbox
      mask CallbackString:
      | |||||||||||fft_callback_arch(gcb);||||% make mutually exclusive with use_embedded.
      | 
      | use_hdl = get_param(gcb, 'use_hdl');
      | if strcmp(use_hdl, 'on'),
      |     set_param_state(gcb, 'use_embedded', 'off');
      | else
      |     set_param_state(gcb, 'use_embedded', 'on');
      | end|% make mutually exclusive with use_hdl.
      | 
      | use_hdl = get_param(gcb, 'use_embedded');
      | if strcmp(use_hdl, 'on'),
      |     set_param_state(gcb, 'use_hdl', 'off');
      | else
      |     set_param_state(gcb, 'use_hdl', 'on');
      | end|hardcode_shifts = get_param(gcb, 'hardcode_shifts');
      | set_param_state(gcb, 'downshift', hardcode_shifts);|fft_callback_dsp48_adders(gcb);
      mask TabNameString: Basic,Basic,Basic,Basic,Basic,Latency,Latency,Latency,Latency,Implementation,Implementation,Implementation,Implementation,Implementation,Implementation,Implementation,Implementation,Implementation,Implementation
  fft_stage_3 : Subsystem  AncestorBlock=casper_library_ffts/fft_stage_n  mask(fft_stage_n){FFTSize=3, FFTStage=3, input_bit_width=8, coeff_bit_width=8, downshift=off, add_latency=2, mult_latency=3, bram_latency=1, conv_latency=1, quantization=Truncate, overflow=Wrap, arch=Virtex5, opt_target=logic, delays_bram=off, coeffs_bram=off, use_hdl=on, use_embedded=off, hardcode_shifts=off, dsp48_adders=on}
      mask prompts: FFTSize "Size of FFT: (2^? pts)"; FFTStage "Stage of FFT:"; input_bit_width "Input/Output Bit Width:"; coeff_bit_width "Coefficient Bit Width"; add_latency "Add Latency"; mult_latency "Mult Latency"; bram_latency "BRAM Latency"; conv_latency "Convert latency"; quantization "Quantization Behavior"; overflow "Overflow Behavior"; arch "Architecture"; opt_target "Use less"; delays_bram "Implement Delays in BRAM"; coeffs_bram "Store Coefficients in BRAM"; use_hdl "Use behavioural HDL for mutlipliers"; use_embedded "Use embedded multipliers"; hardcode_shifts "Hardcode shift schedule"; dsp48_adders "Use DSP48s for adders"
      mask help: FFT internal block.
      mask init: same as fft_biplex_real_4x_dsp48_opt_test/fft_biplex_real_4x/biplex_core/fft_stage_1
      settings: AttributesFormatString=|
      | [3/3]
      | delays in slices
      | coeffs in slices
      mask StyleString: edit,edit,edit,edit,checkbox,edit,edit,edit,edit,popup(Truncate|Round  (unbiased: +/- Inf)|Round  (unbiased: Even Values)),popup(Wrap|Saturate|Error),popup(Virtex2Pro|Virtex5),popup(logic|multipliers),checkbox,checkbox,checkbox,checkbox,checkbox,checkbox
      mask CallbackString:
      | |||||||||||fft_callback_arch(gcb);||||% make mutually exclusive with use_embedded.
      | 
      | use_hdl = get_param(gcb, 'use_hdl');
      | if strcmp(use_hdl, 'on'),
      |     set_param_state(gcb, 'use_embedded', 'off');
      | else
      |     set_param_state(gcb, 'use_embedded', 'on');
      | end|% make mutually exclusive with use_hdl.
      | 
      | use_hdl = get_param(gcb, 'use_embedded');
      | if strcmp(use_hdl, 'on'),
      |     set_param_state(gcb, 'use_hdl', 'off');
      | else
      |     set_param_state(gcb, 'use_hdl', 'on');
      | end|hardcode_shifts = get_param(gcb, 'hardcode_shifts');
      | set_param_state(gcb, 'downshift', hardcode_shifts);|fft_callback_dsp48_adders(gcb);
      mask TabNameString: Basic,Basic,Basic,Basic,Basic,Latency,Latency,Latency,Latency,Implementation,Implementation,Implementation,Implementation,Implementation,Implementation,Implementation,Implementation,Implementation,Implementation
  sync_out : Outport
  out1 : Outport  Port=2
  out2 : Outport  Port=3
  of : Outport  Port=4
  wires:
  fft_stage_1/1(out1) -> fft_stage_2/1(in1)
  fft_stage_1/2(out2) -> fft_stage_2/2(in2)
  fft_stage_1/3(of) -> fft_stage_2/3(of_in)
  fft_stage_1/4(sync_out) -> fft_stage_2/4(sync)
  shift/1 -> fft_stage_2/5(shift), fft_stage_3/5(shift), fft_stage_1/5(shift)
  fft_stage_2/1(out1) -> fft_stage_3/1(in1)
  fft_stage_2/2(out2) -> fft_stage_3/2(in2)
  fft_stage_2/3(of) -> fft_stage_3/3(of_in)
  fft_stage_2/4(sync_out) -> fft_stage_3/4(sync)
  pol1/1 -> fft_stage_1/1(in1)
  pol2/1 -> fft_stage_1/2(in2)
  Constant/1 -> fft_stage_1/3(of_in)
  sync/1 -> fft_stage_1/4(sync)
  fft_stage_3/1(out1) -> out1/1
  fft_stage_3/2(out2) -> out2/1
  fft_stage_3/3(of) -> of/1
  fft_stage_3/4(sync_out) -> sync_out/1

== system fft_biplex_real_4x_dsp48_opt_test/fft_biplex_real_4x/ri_to_c0 ==
  re : Inport  OutDataType=sfix(16)  OutScaling=2^0
  im : Inport  Port=2  OutDataType=sfix(16)  OutScaling=2^0
  concat : xbsIndex_r4/Concat  num_inputs=2  dbl_ovrd=off  block_type=concat
      settings: block_version=9.1.01
  force_im : xbsIndex_r4/Reinterpret  force_arith_type=on  arith_type=Unsigned  force_bin_pt=on  bin_pt=0  block_type=reinterpret
      settings: infoedit="Changes signal type without altering the binary representation.   You can changed the signal between signed and unsigned, and relocate the binary point.<P><P>Hardware notes: In hardware this block costs nothing.<P><P>Example:  Suppose the input is 6 bits wide, signed, with 2 fractional bits, and the output is forced to unsigned with 0 fractional bits.  Then an input of -2.0 (1110.00 in binary 2's complement) becomes an output of 56 (111000 in binary)."  block_version=9.1.01
  force_re : xbsIndex_r4/Reinterpret  force_arith_type=on  arith_type=Unsigned  force_bin_pt=on  bin_pt=0  block_type=reinterpret
      settings: infoedit="Changes signal type without altering the binary representation.   You can changed the signal between signed and unsigned, and relocate the binary point.<P><P>Hardware notes: In hardware this block costs nothing.<P><P>Example:  Suppose the input is 6 bits wide, signed, with 2 fractional bits, and the output is forced to unsigned with 0 fractional bits.  Then an input of -2.0 (1110.00 in binary 2's complement) becomes an output of 56 (111000 in binary)."  block_version=9.1.01
  c : Outport  OutDataType=sfix(16)  OutScaling=2^0
  wires:
  force_re/1 -> concat/1
  force_im/1 -> concat/2
  re/1 -> force_re/1
  concat/1 -> c/1
  im/1 -> force_im/1

== system fft_biplex_real_4x_dsp48_opt_test/fft_biplex_real_4x/ri_to_c1 ==
  re : Inport  OutDataType=sfix(16)  OutScaling=2^0
  im : Inport  Port=2  OutDataType=sfix(16)  OutScaling=2^0
  concat : xbsIndex_r4/Concat  num_inputs=2  dbl_ovrd=off  block_type=concat
      settings: block_version=9.1.01
  force_im : xbsIndex_r4/Reinterpret  force_arith_type=on  arith_type=Unsigned  force_bin_pt=on  bin_pt=0  block_type=reinterpret
      settings: infoedit="Changes signal type without altering the binary representation.   You can changed the signal between signed and unsigned, and relocate the binary point.<P><P>Hardware notes: In hardware this block costs nothing.<P><P>Example:  Suppose the input is 6 bits wide, signed, with 2 fractional bits, and the output is forced to unsigned with 0 fractional bits.  Then an input of -2.0 (1110.00 in binary 2's complement) becomes an output of 56 (111000 in binary)."  block_version=9.1.01
  force_re : xbsIndex_r4/Reinterpret  force_arith_type=on  arith_type=Unsigned  force_bin_pt=on  bin_pt=0  block_type=reinterpret
      settings: infoedit="Changes signal type without altering the binary representation.   You can changed the signal between signed and unsigned, and relocate the binary point.<P><P>Hardware notes: In hardware this block costs nothing.<P><P>Example:  Suppose the input is 6 bits wide, signed, with 2 fractional bits, and the output is forced to unsigned with 0 fractional bits.  Then an input of -2.0 (1110.00 in binary 2's complement) becomes an output of 56 (111000 in binary)."  block_version=9.1.01
  c : Outport  OutDataType=sfix(16)  OutScaling=2^0
  wires:
  force_re/1 -> concat/1
  force_im/1 -> concat/2
  re/1 -> force_re/1
  concat/1 -> c/1
  im/1 -> force_im/1

== system fft_biplex_real_4x_dsp48_opt_test/fft_biplex_real_4x/bi_real_unscr_4x/delay_srl0 ==
  in : Inport  OutDataType=sfix(16)  OutScaling=2^0
  delay_ff : xbsIndex_r4/Delay  en=off  latency=ff_delay  dbl_ovrd=off  reg_retiming=off  block_type=delay
      settings: xl_area=[0, 0, 0, 0, 0, 0, 0]  block_version=9.1.01
  delay_srl : xbsIndex_r4/Delay  en=off  latency=srl_delay  dbl_ovrd=off  reg_retiming=off  block_type=delay
      settings: xl_area=[0, 0, 0, 0, 0, 0, 0]  block_version=9.1.01
  out : Outport  OutDataType=sfix(16)  OutScaling=2^0
  wires:
  delay_ff/1 -> delay_srl/1
  in/1 -> delay_ff/1
  delay_srl/1 -> out/1

== system fft_biplex_real_4x_dsp48_opt_test/fft_biplex_real_4x/bi_real_unscr_4x/delay_srl1 ==
  in : Inport  OutDataType=sfix(16)  OutScaling=2^0
  delay_ff : xbsIndex_r4/Delay  en=off  latency=ff_delay  dbl_ovrd=off  reg_retiming=off  block_type=delay
      settings: xl_area=[0, 0, 0, 0, 0, 0, 0]  block_version=9.1.01
  delay_srl : xbsIndex_r4/Delay  en=off  latency=srl_delay  dbl_ovrd=off  reg_retiming=off  block_type=delay
      settings: xl_area=[0, 0, 0, 0, 0, 0, 0]  block_version=9.1.01
  out : Outport  OutDataType=sfix(16)  OutScaling=2^0
  wires:
  delay_ff/1 -> delay_srl/1
  in/1 -> delay_ff/1
  delay_srl/1 -> out/1

== system fft_biplex_real_4x_dsp48_opt_test/fft_biplex_real_4x/bi_real_unscr_4x/hilbert_dsp48e0 ==
  a : Inport
  b : Inport  Port=2
  Convert{0..3} (4 alike) : xbsIndex_r4/Convert  arith_type="Signed  (2's comp)"  n_bits=BitWidth  bin_pt=BitWidth - 1  quantization="Round  (unbiased: Even Values)"  overflow=Wrap  latency=conv_latency  dbl_ovrd=off  pipeline=off  block_type=convert
      settings: xl_area=[0, 0, 0, 0, 0, 0, 0]
  Scale{0..3} (4 alike) : xbsIndex_r4/Scale  scale_factor=-1  dbl_ovrd=off  block_type=scale
  c_to_ri0 : Subsystem  AncestorBlock=casper_library_misc/c_to_ri  mask(c_to_ri){n_bits=BitWidth, bin_pt=BitWidth-1}
      mask prompts: n_bits "Bit Width"; bin_pt "Binary Point"
      mask help:
      | Outputs real and imaginary components of a complex input.
      | Useful for simplifying interconnects.
      | See also: Real-Imag to Complex (ri_to_c)
      mask init:
      | annotation=sprintf('%d_%d r/i',n_bits,bin_pt);
      | set_param(gcb,'AttributesFormatString',annotation);
      settings: AttributesFormatString=8_7 r/i
      mask Help: eval('xlWeb(''http://casper.berkeley.edu/wiki/C_to_ri'')')
  c_to_ri1 : Subsystem  AncestorBlock=casper_library_ffts_internal/sincos_dsp48e/c_to_ri0  mask(c_to_ri){n_bits=BitWidth, bin_pt=BitWidth-1}
      mask prompts: n_bits "Bit Width"; bin_pt "Binary Point"
      mask help:
      | Outputs real and imaginary components of a complex input.
      | Useful for simplifying interconnects.
      | See also: Real-Imag to Complex (ri_to_c)
      mask init:
      | annotation=sprintf('%d_%d r/i',n_bits,bin_pt);
      | set_param(gcb,'AttributesFormatString',annotation);
      settings: AttributesFormatString=8_7 r/i
      mask Help: eval('xlWeb(''http://casper.berkeley.edu/wiki/C_to_ri'')')
  cadd : Subsystem  AncestorBlock=casper_library_misc/caddsub_dsp48e  mask(caddsub_dsp48e){mode=Addition, n_bits_a=8, bin_pt_a=7, n_bits_b=8, bin_pt_b=7, full_precision=on, n_bits_c=19, bin_pt_c=17, quantization=Truncate, overflow=Wrap, cast_latency=0}
      mask prompts: mode "Operation:"; n_bits_a "Bit width 'a':"; bin_pt_a "Binary point 'a':"; n_bits_b "Bit width 'b':"; bin_pt_b "Binary point 'b':"; full_precision "Full precision"; n_bits_c "Bit width out:"; bin_pt_c "Binary point out:"; cast_latency "Cast Latency:"
      mask help:
      | Adds or subtracts two complex numbers using a DSP48E.
      |
      | The two inputs can have different bit widths and binary points, but their sum cannot exceed 24 bits.
      mask init:
      | caddsub_dsp48e_init(gcb, ...
      |     'mode', mode, ...
      |     'n_bits_a', n_bits_a, ...
      |     'bin_pt_a', bin_pt_a, ...
      |     'n_bits_b', n_bits_b, ...
      |     'bin_pt_b', bin_pt_b, ...
      |     'full_precision', full_precision, ...
      |     'n_bits_c', n_bits_c, ...
      |     'bin_pt_c', bin_pt_c, ...
      |     'quantization', quantization, ...
      |     'overflow', overflow, ...
      |     'cast_latency', cast_latency);
      settings: AttributesFormatString=|
      | 8_7 + 8_7 ==> 9_7
      | Mode=Addition
      | Latency=2
      mask StyleString: popup(Addition|Subtraction),edit,edit,edit,edit,checkbox,edit,edit,popup(Truncate|Round  (unbiased: +/- Inf)|Round  (unbiased: Even Values)),popup(Wrap|Saturate|Flag as error),edit
      mask CallbackString:
      | |||||thisVariable = 'full_precision';
      | affectedVars = { ...
      |     'n_bits_c', ...
      |     'bin_pt_c', ...
      |     'quantization', ...
      |     'overflow', ...
      |     'cast_latency', ...
      | };
      | 
      | thisBlock = gcb();
      | thisVarState = get_param(thisBlock, thisVariable);
      | maskNames = get_param(thisBlock, 'MaskNames');
      | maskEnables = get_param(thisBlock, 'MaskEnables');
      | 
      | if strcmp(thisVarState, 'on'),
      |     targVarState = 'off';
      | else,
      |     targVarState = 'on';
      | end
      | 
      | for varName = affectedVars
      |     varIndex = find(ismember(maskNames, varName));
      |     maskEnables{varIndex} = targVarState;
      | end
      | 
      | set_param(thisBlock, 'MaskEnables', maskEnables);|||||
      mask TabNameString: Basic,Basic,Basic,Basic,Basic,Output Type,Output Type,Output Type,Output Type,Output Type,Output Type
  csub : Subsystem  AncestorBlock=casper_library_misc/caddsub_dsp48e  mask(caddsub_dsp48e){mode=Subtraction, n_bits_a=8, bin_pt_a=7, n_bits_b=8, bin_pt_b=7, full_precision=on, n_bits_c=19, bin_pt_c=17, quantization=Truncate, overflow=Wrap, cast_latency=0}
      mask prompts: mode "Operation:"; n_bits_a "Bit width 'a':"; bin_pt_a "Binary point 'a':"; n_bits_b "Bit width 'b':"; bin_pt_b "Binary point 'b':"; full_precision "Full precision"; n_bits_c "Bit width out:"; bin_pt_c "Binary point out:"; cast_latency "Cast Latency:"
      mask help:
      | Adds or subtracts two complex numbers using a DSP48E.
      |
      | The two inputs can have different bit widths and binary points, but their sum cannot exceed 24 bits.
      mask init: same as fft_biplex_real_4x_dsp48_opt_test/fft_biplex_real_4x/bi_real_unscr_4x/hilbert_dsp48e0/cadd
      settings: AttributesFormatString=|
      | 8_7 + 8_7 ==> 9_7
      | Mode=Subtraction
      | Latency=2
      mask StyleString: popup(Addition|Subtraction),edit,edit,edit,edit,checkbox,edit,edit,popup(Truncate|Round  (unbiased: +/- Inf)|Round  (unbiased: Even Values)),popup(Wrap|Saturate|Flag as error),edit
      mask CallbackString:
      | |||||thisVariable = 'full_precision';
      | affectedVars = { ...
      |     'n_bits_c', ...
      |     'bin_pt_c', ...
      |     'quantization', ...
      |     'overflow', ...
      |     'cast_latency', ...
      | };
      | 
      | thisBlock = gcb();
      | thisVarState = get_param(thisBlock, thisVariable);
      | maskNames = get_param(thisBlock, 'MaskNames');
      | maskEnables = get_param(thisBlock, 'MaskEnables');
      | 
      | if strcmp(thisVarState, 'on'),
      |     targVarState = 'off';
      | else,
      |     targVarState = 'on';
      | end
      | 
      | for varName = affectedVars
      |     varIndex = find(ismember(maskNames, varName));
      |     maskEnables{varIndex} = targVarState;
      | end
      | 
      | set_param(thisBlock, 'MaskEnables', maskEnables);|||||
      mask TabNameString: Basic,Basic,Basic,Basic,Basic,Output Type,Output Type,Output Type,Output Type,Output Type,Output Type
  ri_to_c0 : Subsystem  AncestorBlock=casper_library_misc/ri_to_c
      mask Type: ri_to_c
      mask Description:
      | Concatenates real and imaginary inputs into a complex output.
      | Useful for simplifying interconnects.
      | See also: Complex to Real-Imag (c_to_ri)
      mask Help: eval('xlWeb(''http://casper.berkeley.edu/wiki/Ri_to_c'')')
  ri_to_c1 : Subsystem  AncestorBlock=casper_library_misc/ri_to_c
      mask Type: ri_to_c
      mask Description:
      | Concatenates real and imaginary inputs into a complex output.
      | Useful for simplifying interconnects.
      | See also: Complex to Real-Imag (c_to_ri)
      mask Help: eval('xlWeb(''http://casper.berkeley.edu/wiki/Ri_to_c'')')
  even : Outport
  odd : Outport  Port=2
  wires:
  c_to_ri1/2(im) -> cadd/4(b_im), csub/3(b_re)
  Convert3/1 -> ri_to_c1/2(im)
  Convert1/1 -> ri_to_c1/1(re)
  Convert2/1 -> ri_to_c0/2(im)
  c_to_ri0/2(im) -> cadd/2(a_im), csub/1(a_re)
  Convert0/1 -> ri_to_c0/1(re)
  c_to_ri1/1(re) -> csub/2(a_im), cadd/3(b_re)
  Scale3/1 -> Convert3/1
  Scale2/1 -> Convert2/1
  Scale1/1 -> Convert1/1
  Scale0/1 -> Convert0/1
  csub/2(c_im) -> Scale3/1
  csub/1(c_re) -> Scale2/1
  ri_to_c0/1(c) -> even/1
  ri_to_c1/1(c) -> odd/1
  cadd/2(c_im) -> Scale1/1
  cadd/1(c_re) -> Scale0/1
  c_to_ri0/1(re) -> csub/4(b_im), cadd/1(a_re)
  b/1 -> c_to_ri1/1(c)
  a/1 -> c_to_ri0/1(c)
